simulink model "pfb_fft_d3a"  (R2021a)
settings: Solver=VariableStepAuto  StartTime=0.0  StopTime=100.0  RelTol=1e-3
undefined symbols (not defined in the file): i, pfb_coeff_gen_calc
libraries: xbsIndex_r4 x11529, casper_library_misc x39, casper_library_delays x39, xbsReplacements_r4 x2
(part 1 of 118)
settings Model: Creator=tbuser  LastModifiedBy=ih

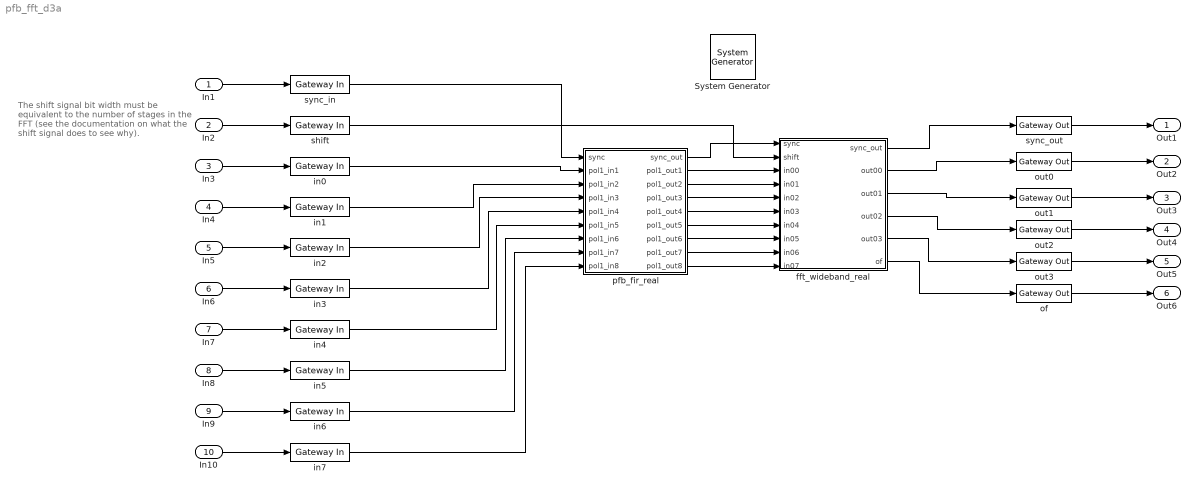
== system pfb_fft_d3a ==
  note: The shift signal bit width must be equivalent to the number of stages in the FFT (see the documentation on what the shift signal does to see why).
  In1 : Inport
  In2 : Inport  Port=2
  In3 : Inport  Port=3
  In4 : Inport  Port=4
  In5 : Inport  Port=5
  In6 : Inport  Port=6
  In7 : Inport  Port=7
  In8 : Inport  Port=8
  In9 : Inport  Port=9
  In10 : Inport  Port=10
  " System Generator" : xbsIndex_r4/ System Generator  Tag=genX  xilinxfamily=zynquplusRFSOC  part=xczu48dr  speed=-1-i  package=ffvg1517  synthesis_tool=Vivado  clock_wrapper=Clock Enables  directory=/home/ih/casper/pfb_fft_d3a  proj_type=Vivado  Synth_file=Vivado Synthesis Defaults  Impl_file=Vivado Implementation Defaults  testbench=off  simulink_period=1  sysclk_period=2.5  dcm_input_clock_period=10  incr_netlist=off  trim_vbits=Everywhere in SubSystem  dbl_ovrd=According to Block Masks  core_generation=According to Block Masks  run_coregen=off  deprecated_control=off  eval_field=0  block_type=sysgen
  fft_wideband_real : Subsystem  Tag=casper:fft_wideband_real  AncestorBlock=casper_library_ffts/fft_wideband_real  mask(fft_wideband_real){n_streams=1, FFTSize=14, n_inputs=3, input_bit_width=18, bin_pt_in=17, coeff_bit_width=18, unscramble=on, async=off, floating_point=off, float_type=single, exp_width=8, frac_width=24, add_latency=1, mult_latency=2, bram_latency=2, conv_latency=1, input_latency=0, biplex_direct_latency=0, add_pipe_latency=0, mult_pipe_latency=0, quantization=Round  (unbiased: Even Values), overflow=Wrap, delays_bit_limit=9, coeffs_bit_limit=9, coeff_sharing=on, coeff_decimation=on, coeff_generation=on, cal_bits=1, n_bits_rotation=25, mult_spec=2, max_fanout=4, bitgrowth=off, max_bits=18, hardcode_shifts=off, shift_schedule=[], dsp48_adders=off}
      mask prompts: n_streams "Number simultaneous streams"; FFTSize "Size of FFT: (2^? pts)"; n_inputs "Number of Simultaneous Inputs: (2^?)"; input_bit_width "Input Bit Width"; bin_pt_in "Input binary point"; coeff_bit_width "Coefficient Bit Width"; unscramble "Unscramble output (ie, put channels in canonical order)"; async "Asynchronous operation"; floating_point "floating point"; float_type "float type"; exp_width "exponent width"; frac_width "fraction width"; add_latency "Add Latency"; mult_latency "Mult Latency"; bram_latency "BRAM Latency"; conv_latency "Convert Latency"; input_latency "Input Latency"; biplex_direct_latency "Latency between biplexes and fft_direct"; add_pipe_latency "Add Interface Pipeline Latency"; mult_pipe_latency "CMult Pipeline Latency"; quantization "Quantization Behavior"; overflow "Overflow Behavior"; delays_bit_limit "Number bits above which to store stage's delays in BRAM (2^? bits)"; coeffs_bit_limit "Number bits above which to store stage's coefficients in BRAM (2^? bits)"; coeff_sharing "BRAM sharing in coeff storage"; coeff_decimation "Store a fraction of coeff factors where useful"; coeff_generation "Generate coeffs with multipliers where useful"; cal_bits "Number calibration locations when generating coeffs (2^?)"; n_bits_rotation "Feedback rotation vector resolution"; mult_spec "Multiplier impl. (0=core, 1=embedded, 2=behavioural) (left=1st stage, or just one value)"; max_fanout "Maximum fanout"; bitgrowth "Bitgrowth instead of shifting"; max_bits "Max bits to grow to"; hardcode_shifts "Hardcode shift schedule"; shift_schedule "Shift schedule"; dsp48_adders "DSP48 adders in butterfly"
      mask help: A real-sampled wideband FFT.
      mask init:
      | fft_wideband_real_init(gcb, ...
      |     'n_streams', n_streams, ...
      |     'FFTSize', FFTSize, ...
      |     'n_inputs', n_inputs, ...
      |     'input_bit_width', input_bit_width, ...
      |     'bin_pt_in', bin_pt_in, ...
      |     'coeff_bit_width', coeff_bit_width, ...
      |     'floating_point', floating_point, ...
      |     'float_type', float_type, ...
      |     'exp_width', exp_width, ...
      |     'frac_width', frac_width, ...
      |     'unscramble', unscramble, ...
      |     'async', async, ...
      |     'add_latency', add_latency, ...
      |     'mult_latency', mult_latency, ...
      |     'bram_latency', bram_latency, ...
      |     'conv_latency', conv_latency, ...
      |     'input_latency', input_latency, ...
      |     'add_pipe_latency', add_pipe_latency, ...
      |     'mult_pipe_latency', mult_pipe_latency, ...
      |     'biplex_direct_latency', biplex_direct_latency, ...
      |     'quantization', quantization, ...
      |     'overflow', overflow, ...
      |     'delays_bit_limit', delays_bit_limit, ...
      |     'coeffs_bit_limit', coeffs_bit_limit, ...
      |     'coeff_sharing', coeff_sharing, ...
      |     'coeff_decimation', coeff_decimation, ...
      |     'coeff_generation', coeff_generation, ...
      |     'cal_bits', cal_bits, ...
      |     'n_bits_rotation', n_bits_rotation, ...
      |     'max_fanout', max_fanout, ...   
      |     'mult_spec', mult_spec, ...
      |     'bitgrowth', bitgrowth, ...
      |     'max_bits', max_bits, ...
      |     'hardcode_shifts', hardcode_shifts, ...
      |     'shift_schedule', shift_schedule, ...
      |     'dsp48_adders', dsp48_adders);
      settings: AttributesFormatString=|
      | 14 stages
      | (18,18)
      | Round  (unbiased: Even Values)
      | Wrap
      mask Help: eval('xlWeb(''http://casper.berkeley.edu/wiki/Fft_wideband_real'')')
      mask Callback floating_point:
      | onoff = get_param(gcb, 'floating_point');
      | if strcmp(onoff,'on')
      |     enable_fixpt = 'off';
      |     set_param_state(gcb, 'float_type', 'on')
      | 
      |     f_type = get_param(gcb, 'float_type')
      |     if strcmp(f_type,'custom')
      |         set_param_state(gcb, 'exp_width', 'on')
      |         set_param_state(gcb, 'frac_width', 'on')
      |     else
      |         set_param_state(gcb, 'exp_width', 'off')
      |         set_param_state(gcb, 'frac_width', 'off')
      |     end
      | 
      | 
      | else
      |     enable_fixpt = 'on';
      |     set_param_state(gcb, 'float_type', 'off')
      |     set_param_state(gcb, 'exp_width', 'off')
      |     set_param_state(gcb, 'frac_width', 'off')
      | end
      | 
      | set_param_state(gcb, 'input_bit_width', enable_fixpt)
      | set_param_state(gcb, 'bin_pt_in', enable_fixpt)
      | set_param_state(gcb, 'coeff_bit_width', enable_fixpt)
      mask TypeOptions float_type: single | custom
      mask Callback float_type:
      | f_type = get_param(gcb, 'float_type');
      | if strcmp(f_type,'custom')
      |     set_param_state(gcb, 'exp_width', 'on')
      |     set_param_state(gcb, 'frac_width', 'on')
      | else
      |     set_param_state(gcb, 'exp_width', 'off')
      |     set_param_state(gcb, 'frac_width', 'off')
      | end
      mask TypeOptions quantization: Truncate | Round  (unbiased: +/- Inf) | Round  (unbiased: Even Values)
      mask TypeOptions overflow: Wrap | Saturate | Error
      mask Callback hardcode_shifts:
      | hardcode_shifts = get_param(gcb, 'hardcode_shifts');
      | set_param_state(gcb, 'shift_schedule', hardcode_shifts);
      mask Callback dsp48_adders: fft_callback_dsp48_adders(gcb);
      mask DialogControl ParameterTabVar0 Prompt: Basic
      mask DialogControl ParameterTabVar01 Prompt: Latency
      mask DialogControl ParameterTabVar012 Prompt: Implementation
  in{0..7} (8 alike) : xbsIndex_r4/Gateway In  gui_display_data_type=Fixed-point  arith_type="Signed  (2's comp)"  n_bits=14  bin_pt=0  preci_type=Single  exp_width=8  frac_width=24  rows=1  columns=1  quantization="Round  (unbiased: +/- Inf)"  overflow=Saturate  period=1  UseAsADC=off  ADCChannel='1'  interface=None  automatic_assignment=on  address_offset=hex2dec('00')  intf_name=''  intf_description=''  default_value=0  timing_constraint=None  locs_specified=off  LOCs={}  io_standard={}  inherit_from_input=off  hdl_port=on  dbl_ovrd=off  block_type=gatewayin
  of : xbsIndex_r4/Gateway Out  inherit_from_input=off  hdl_port=on  rows=1  columns=1  UseAsDAC=off  DACChannel='1'  interface=None  automatic_assignment=on  address_offset=hex2dec('00')  intf_name=''  intf_description=''  timing_constraint=None  locs_specified=off  LOCs={}  io_standard={}  block_type=gatewayout
  out{0..3} (4 alike) : xbsIndex_r4/Gateway Out  inherit_from_input=on  hdl_port=on  rows=1  columns=1  UseAsDAC=off  DACChannel='1'  interface=None  automatic_assignment=on  address_offset=hex2dec('00')  intf_name=''  intf_description=''  timing_constraint=None  locs_specified=off  LOCs={}  io_standard={}  block_type=gatewayout
  pfb_fir_real : Subsystem  Tag=casper:pfb_fir_real  AncestorBlock=casper_library_pfbs/pfb_fir_real  mask(pfb_fir_real){PFBSize=14, TotalTaps=4, WindowType=hamming, n_inputs=3, n_pol_blocks=1, MakeBiplex=off, BitWidthIn=14, BitWidthOut=18, CoeffBitWidth=18, CoeffDistMem=off, add_latency=1, mult_latency=2, bram_latency=2, fan_latency=1, conv_latency=1, quantization=Round  (unbiased: Even Values), fwidth=1, mult_spec=2, adder_folding=on, adder_imp=Fabric, coeffs_share=off}
      mask prompts: PFBSize "Size of PFB: (2^? pnts)"; TotalTaps "Total Number of Taps:"; WindowType "Windowing Function:"; n_inputs "Number of Simultaneous Inputs: (2^?)"; n_pol_blocks "Number of independent input streams (I.e., number of different polarizations)"; MakeBiplex "Make Biplex?"; BitWidthIn "Input Bitwidth:"; BitWidthOut "Output Bitwidth:"; CoeffBitWidth "Coefficient Bitwidth:"; CoeffDistMem "Use Distributed Memory for Coeffs"; add_latency "Add Latency"; mult_latency "Mult Latency"; bram_latency "BRAM Latency"; fan_latency "Fanout latency"; conv_latency "Convert latency"; quantization "Quantization Behavior"; fwidth "Bin Width Scaling (normal=1)"; mult_spec "Multiplier specification (0=core, 1=embedded, 2=behavioural) (left=1st tap, or just one value)"; adder_folding "Fold adders into DSPs"; adder_imp "Adder implementation"; coeffs_share "Share coefficients between polarisations (use less BRAM)?"
      mask help:
      | Fold adders into DSPs: Causes adders to be absorbed into DSP blocks (supported in Virtex5)
      | Adder implementation: Cores using Fabric or DSP48 or behavioral HDL
      mask init:
      | pfb_fir_real_init(gcb, ...
      |     'PFBSize', PFBSize, ...
      |     'TotalTaps', TotalTaps, ...
      |     'WindowType', WindowType, ...
      |     'n_inputs', n_inputs, ...
      |     'MakeBiplex', MakeBiplex, ...
      |     'BitWidthIn', BitWidthIn, ...
      |     'BitWidthOut', BitWidthOut, ...
      |     'CoeffBitWidth', CoeffBitWidth, ...
      |     'CoeffDistMem', CoeffDistMem, ...
      |     'add_latency', add_latency, ...
      |     'mult_latency', mult_latency, ...
      |     'bram_latency', bram_latency, ...
      |     'fan_latency', fan_latency, ...
      |     'conv_latency', conv_latency, ...
      |     'quantization', quantization, ...
      |     'fwidth', fwidth, ...
      |     'mult_spec', mult_spec, ...
      |     'adder_folding', adder_folding, ...
      |     'adder_imp', adder_imp, ...
      |     'coeffs_share', coeffs_share);
      settings: AttributesFormatString=taps=4, add_latency=1
      mask Help: eval('xlWeb(''http://casper.berkeley.edu/wiki/Pfb_fir_real'')')
      mask Callback TotalTaps:
      | %num_taps = eval(get_param(gcb, 'TotalTaps'));
      | %old_vec = eval(get_param(gcb, 'mult_spec'));=-0l
      | 
      | %vec = 2.*ones(1,num_taps);
      | %old_size = length(old_vec);
      | 
      | %if(old_size <= num_taps),
      | %    new_size = old_size;
      | %else,
      | %    new_size = num_taps;
      | %end
      | 
      | %for n = 1:new_size, vec(n) = old_vec(n); end
      | %set_param(gcb, 'mult_spec', mat2str(vec));
      mask TypeOptions WindowType: bartlett | barthannwin | blackman | blackmanharris | bohamwin | chebwin | flattopwin | gausswin | hamming | hann | kaiser | nuttallwin | parzenwin | rectwin | tukeywin | triang | userwindow
      mask TypeOptions quantization: Truncate | Round  (unbiased: +/- Inf) | Round  (unbiased: Even Values)
      mask TypeOptions adder_imp: Behavioral | Fabric | DSP48
  shift : xbsIndex_r4/Gateway In  gui_display_data_type=Fixed-point  arith_type=Unsigned  n_bits=14  bin_pt=0  preci_type=Single  exp_width=8  frac_width=24  rows=1  columns=1  quantization="Round  (unbiased: +/- Inf)"  overflow=Saturate  period=1  UseAsADC=off  ADCChannel='1'  interface=None  automatic_assignment=on  address_offset=hex2dec('00')  intf_name=''  intf_description=''  default_value=0  timing_constraint=None  locs_specified=off  LOCs={}  io_standard={}  inherit_from_input=off  hdl_port=on  dbl_ovrd=off  block_type=gatewayin
  sync_in : xbsIndex_r4/Gateway In  gui_display_data_type=Boolean  arith_type=Boolean  n_bits=16  bin_pt=14  preci_type=Single  exp_width=8  frac_width=24  rows=1  columns=1  quantization="Round  (unbiased: +/- Inf)"  overflow=Saturate  period=1  UseAsADC=off  ADCChannel='1'  interface=None  automatic_assignment=on  address_offset=hex2dec('00')  intf_name=''  intf_description=''  default_value=0  timing_constraint=None  locs_specified=off  LOCs={}  io_standard={}  inherit_from_input=off  hdl_port=on  dbl_ovrd=off  block_type=gatewayin
  sync_out : xbsIndex_r4/Gateway Out  inherit_from_input=off  hdl_port=on  rows=1  columns=1  UseAsDAC=off  DACChannel='1'  interface=None  automatic_assignment=on  address_offset=hex2dec('00')  intf_name=''  intf_description=''  timing_constraint=None  locs_specified=off  LOCs={}  io_standard={}  block_type=gatewayout
  Out1 : Outport
  Out2 : Outport  Port=2
  Out3 : Outport  Port=3
  Out4 : Outport  Port=4
  Out5 : Outport  Port=5
  Out6 : Outport  Port=6
  wires:
  fft_wideband_real/1(sync_out) -> sync_out/1
  fft_wideband_real/2(out00) -> out0/1
  fft_wideband_real/3(out01) -> out1/1
  fft_wideband_real/6(of) -> of/1
  fft_wideband_real/4(out02) -> out2/1
  fft_wideband_real/5(out03) -> out3/1
  pfb_fir_real/2(pol1_out1) -> fft_wideband_real/3(in00)
  pfb_fir_real/3(pol1_out2) -> fft_wideband_real/4(in01)
  pfb_fir_real/4(pol1_out3) -> fft_wideband_real/5(in02)
  pfb_fir_real/5(pol1_out4) -> fft_wideband_real/6(in03)
  pfb_fir_real/6(pol1_out5) -> fft_wideband_real/7(in04)
  pfb_fir_real/7(pol1_out6) -> fft_wideband_real/8(in05)
  pfb_fir_real/8(pol1_out7) -> fft_wideband_real/9(in06)
  pfb_fir_real/9(pol1_out8) -> fft_wideband_real/10(in07)
  shift/1 -> fft_wideband_real/2(shift)
  sync_in/1 -> pfb_fir_real/1(sync)
  pfb_fir_real/1(sync_out) -> fft_wideband_real/1(sync)
  in0/1 -> pfb_fir_real/2(pol1_in1)
  in1/1 -> pfb_fir_real/3(pol1_in2)
  in2/1 -> pfb_fir_real/4(pol1_in3)
  in3/1 -> pfb_fir_real/5(pol1_in4)
  in4/1 -> pfb_fir_real/6(pol1_in5)
  in5/1 -> pfb_fir_real/7(pol1_in6)
  in6/1 -> pfb_fir_real/8(pol1_in7)
  in7/1 -> pfb_fir_real/9(pol1_in8)
  In1/1 -> sync_in/1
  In2/1 -> shift/1
  In3/1 -> in0/1
  In4/1 -> in1/1
  In5/1 -> in2/1
  In6/1 -> in3/1
  In7/1 -> in4/1
  In8/1 -> in5/1
  In9/1 -> in6/1
  In10/1 -> in7/1
  sync_out/1 -> Out1/1
  out0/1 -> Out2/1
  out1/1 -> Out3/1
  out2/1 -> Out4/1
  out3/1 -> Out5/1
  of/1 -> Out6/1

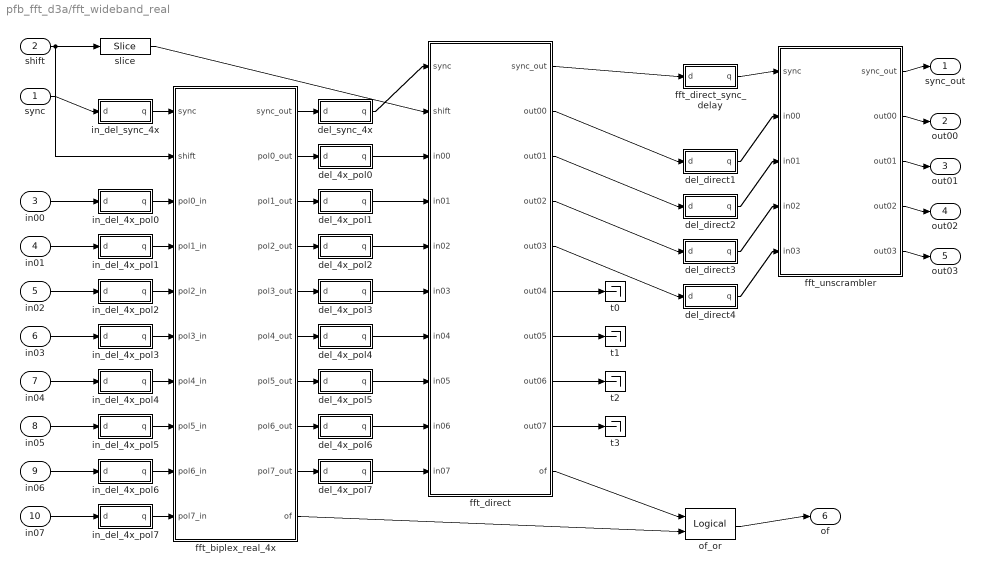
== system pfb_fft_d3a/fft_wideband_real ==
  sync : Inport
  shift : Inport  Port=2
  in00 : Inport  Port=3
  in01 : Inport  Port=4
  in02 : Inport  Port=5
  in03 : Inport  Port=6
  in04 : Inport  Port=7
  in05 : Inport  Port=8
  in06 : Inport  Port=9
  in07 : Inport  Port=10
  del_4x_pol0 : Subsystem  AncestorBlock=casper_library_delays/pipeline  mask(pipeline){csp_latency=0}
      mask prompts: csp_latency "Latency"
      mask help:
      | An explicitly laid-out delay line to avoid mapping to SRL16s
      | for use in pipelining to help achieve timing closure.
      mask init:
      | pipeline_init(gcb,'latency',csp_latency);
      settings: AttributesFormatString=Latency = %<latency>
      mask Display:
      | port_label('input', 1, 'd');
      | port_label('output', 1, 'q');
      | disp(['Z^-', num2str(csp_latency)]);
  del_4x_pol1 : Subsystem  AncestorBlock=casper_library_delays/pipeline  mask(pipeline){csp_latency=0}
      mask prompts: csp_latency "Latency"
      mask help:
      | An explicitly laid-out delay line to avoid mapping to SRL16s
      | for use in pipelining to help achieve timing closure.
      mask init:
      | pipeline_init(gcb,'latency',csp_latency);
      settings: AttributesFormatString=Latency = %<latency>
      mask Display:
      | port_label('input', 1, 'd');
      | port_label('output', 1, 'q');
      | disp(['Z^-', num2str(csp_latency)]);
  del_4x_pol2 : Subsystem  AncestorBlock=casper_library_delays/pipeline  mask(pipeline){csp_latency=0}
      mask prompts: csp_latency "Latency"
      mask help:
      | An explicitly laid-out delay line to avoid mapping to SRL16s
      | for use in pipelining to help achieve timing closure.
      mask init:
      | pipeline_init(gcb,'latency',csp_latency);
      settings: AttributesFormatString=Latency = %<latency>
      mask Display:
      | port_label('input', 1, 'd');
      | port_label('output', 1, 'q');
      | disp(['Z^-', num2str(csp_latency)]);
  del_4x_pol3 : Subsystem  AncestorBlock=casper_library_delays/pipeline  mask(pipeline){csp_latency=0}
      mask prompts: csp_latency "Latency"
      mask help:
      | An explicitly laid-out delay line to avoid mapping to SRL16s
      | for use in pipelining to help achieve timing closure.
      mask init:
      | pipeline_init(gcb,'latency',csp_latency);
      settings: AttributesFormatString=Latency = %<latency>
      mask Display:
      | port_label('input', 1, 'd');
      | port_label('output', 1, 'q');
      | disp(['Z^-', num2str(csp_latency)]);
  del_4x_pol4 : Subsystem  AncestorBlock=casper_library_delays/pipeline  mask(pipeline){csp_latency=0}
      mask prompts: csp_latency "Latency"
      mask help:
      | An explicitly laid-out delay line to avoid mapping to SRL16s
      | for use in pipelining to help achieve timing closure.
      mask init:
      | pipeline_init(gcb,'latency',csp_latency);
      settings: AttributesFormatString=Latency = %<latency>
      mask Display:
      | port_label('input', 1, 'd');
      | port_label('output', 1, 'q');
      | disp(['Z^-', num2str(csp_latency)]);
  del_4x_pol5 : Subsystem  AncestorBlock=casper_library_delays/pipeline  mask(pipeline){csp_latency=0}
      mask prompts: csp_latency "Latency"
      mask help:
      | An explicitly laid-out delay line to avoid mapping to SRL16s
      | for use in pipelining to help achieve timing closure.
      mask init:
      | pipeline_init(gcb,'latency',csp_latency);
      settings: AttributesFormatString=Latency = %<latency>
      mask Display:
      | port_label('input', 1, 'd');
      | port_label('output', 1, 'q');
      | disp(['Z^-', num2str(csp_latency)]);
  del_4x_pol6 : Subsystem  AncestorBlock=casper_library_delays/pipeline  mask(pipeline){csp_latency=0}
      mask prompts: csp_latency "Latency"
      mask help:
      | An explicitly laid-out delay line to avoid mapping to SRL16s
      | for use in pipelining to help achieve timing closure.
      mask init:
      | pipeline_init(gcb,'latency',csp_latency);
      settings: AttributesFormatString=Latency = %<latency>
      mask Display:
      | port_label('input', 1, 'd');
      | port_label('output', 1, 'q');
      | disp(['Z^-', num2str(csp_latency)]);
  del_4x_pol7 : Subsystem  AncestorBlock=casper_library_delays/pipeline  mask(pipeline){csp_latency=0}
      mask prompts: csp_latency "Latency"
      mask help:
      | An explicitly laid-out delay line to avoid mapping to SRL16s
      | for use in pipelining to help achieve timing closure.
      mask init:
      | pipeline_init(gcb,'latency',csp_latency);
      settings: AttributesFormatString=Latency = %<latency>
      mask Display:
      | port_label('input', 1, 'd');
      | port_label('output', 1, 'q');
      | disp(['Z^-', num2str(csp_latency)]);
  del_direct1 : Subsystem  AncestorBlock=casper_library_delays/pipeline  mask(pipeline){csp_latency=0}
      mask prompts: csp_latency "Latency"
      mask help:
      | An explicitly laid-out delay line to avoid mapping to SRL16s
      | for use in pipelining to help achieve timing closure.
      mask init:
      | pipeline_init(gcb,'latency',csp_latency);
      settings: AttributesFormatString=Latency = %<latency>
      mask Display:
      | port_label('input', 1, 'd');
      | port_label('output', 1, 'q');
      | disp(['Z^-', num2str(csp_latency)]);
  del_direct2 : Subsystem  AncestorBlock=casper_library_delays/pipeline  mask(pipeline){csp_latency=0}
      mask prompts: csp_latency "Latency"
      mask help:
      | An explicitly laid-out delay line to avoid mapping to SRL16s
      | for use in pipelining to help achieve timing closure.
      mask init:
      | pipeline_init(gcb,'latency',csp_latency);
      settings: AttributesFormatString=Latency = %<latency>
      mask Display:
      | port_label('input', 1, 'd');
      | port_label('output', 1, 'q');
      | disp(['Z^-', num2str(csp_latency)]);
  del_direct3 : Subsystem  AncestorBlock=casper_library_delays/pipeline  mask(pipeline){csp_latency=0}
      mask prompts: csp_latency "Latency"
      mask help:
      | An explicitly laid-out delay line to avoid mapping to SRL16s
      | for use in pipelining to help achieve timing closure.
      mask init:
      | pipeline_init(gcb,'latency',csp_latency);
      settings: AttributesFormatString=Latency = %<latency>
      mask Display:
      | port_label('input', 1, 'd');
      | port_label('output', 1, 'q');
      | disp(['Z^-', num2str(csp_latency)]);
  del_direct4 : Subsystem  AncestorBlock=casper_library_delays/pipeline  mask(pipeline){csp_latency=0}
      mask prompts: csp_latency "Latency"
      mask help:
      | An explicitly laid-out delay line to avoid mapping to SRL16s
      | for use in pipelining to help achieve timing closure.
      mask init:
      | pipeline_init(gcb,'latency',csp_latency);
      settings: AttributesFormatString=Latency = %<latency>
      mask Display:
      | port_label('input', 1, 'd');
      | port_label('output', 1, 'q');
      | disp(['Z^-', num2str(csp_latency)]);
  del_sync_4x : Subsystem  AncestorBlock=casper_library_delays/pipeline  mask(pipeline){csp_latency=0}
      mask prompts: csp_latency "Latency"
      mask help:
      | An explicitly laid-out delay line to avoid mapping to SRL16s
      | for use in pipelining to help achieve timing closure.
      mask init:
      | pipeline_init(gcb,'latency',csp_latency);
      settings: AttributesFormatString=Latency = %<latency>
      mask Display:
      | port_label('input', 1, 'd');
      | port_label('output', 1, 'q');
      | disp(['Z^-', num2str(csp_latency)]);
  fft_biplex_real_4x : Subsystem  Tag=casper:fft_biplex_real_4x  AncestorBlock=casper_library_ffts/fft_biplex_real_4x  mask(fft_biplex_real_4x){n_inputs=2, FFTSize=11, input_bit_width=18, bin_pt_in=17, coeff_bit_width=18, async=off, floating_point=off, float_type=single, exp_width=8, frac_width=24, add_latency=1, mult_latency=2, bram_latency=2, conv_latency=1, add_pipe_latency=0, mult_pipe_latency=0, quantization=Round  (unbiased: Even Values), overflow=Wrap, delays_bit_limit=9, coeffs_bit_limit=9, coeff_sharing=on, coeff_decimation=on, max_fanout=4, mult_spec=[2 2 2 2 2 2 2 2 2 2 2], bitgrowth=off, max_bits=18, hardcode_shifts=off, shift_schedule=[1 1 1 1 1 1 1 1 1 1 1], dsp48_adders=off}
      mask prompts: n_inputs "Number simultaneous inputs (4*?)"; FFTSize "Size of FFT: (2^? pts)"; input_bit_width "Input bit width"; bin_pt_in "Input binary point"; coeff_bit_width "Coefficient Bit Width"; async "Asynchronous operation"; floating_point "floating point"; float_type "float type"; exp_width "exponent width"; frac_width "fraction width"; add_latency "Add Latency"; mult_latency "Mult Latency"; bram_latency "BRAM Latency"; conv_latency "Convert latency"; add_pipe_latency "Add Interface Pipeline Latency"; mult_pipe_latency "CMult Pipeline Latency"; quantization "Quantization Behavior"; overflow "Overflow Behavior"; delays_bit_limit "Number bits above which to implement stage's delays in BRAM (2^? bits)"; coeffs_bit_limit "Number bits above which to store stage's coefficients in BRAM (2^? bits)"; coeff_sharing "BRAM sharing in coeff storage"; coeff_decimation "Store a fraction of coeff factors where useful"; max_fanout "Maximum fanout"; mult_spec "Multiplier impl. (0=core, 1=embedded, 2=behavioural) (left=1st stage, or just one value)"; bitgrowth "Bitgrowth instead of shifting"; max_bits "Max bits to grow to"; hardcode_shifts "Hardcode shift schedule"; shift_schedule "Shift schedule"; dsp48_adders "DSP48 adders in butterfly"
      mask help: A real-sampled biplex FFT, with output demuxed by 4.
      mask init:
      | fft_biplex_real_4x_init(gcb, ...
      |     'n_inputs', n_inputs, ...
      |     'FFTSize', FFTSize, ...
      |     'input_bit_width', input_bit_width, ...
      |     'bin_pt_in', bin_pt_in, ...
      |     'coeff_bit_width', coeff_bit_width, ...
      |     'floating_point', floating_point, ...
      |     'float_type', float_type, ...
      |     'exp_width', exp_width, ...
      |     'frac_width', frac_width, ...    
      |     'async', async, ...
      |     'add_latency', add_latency, ...
      |     'mult_latency', mult_latency, ...
      |     'bram_latency', bram_latency, ...
      |     'conv_latency', conv_latency, ...
      |     'add_pipe_latency', add_pipe_latency, ...
      |     'mult_pipe_latency', mult_pipe_latency, ...    
      |     'quantization', quantization, ...
      |     'overflow', overflow, ...
      |     'delays_bit_limit', delays_bit_limit, ... 
      |     'coeffs_bit_limit', coeffs_bit_limit, ...
      |     'coeff_sharing', coeff_sharing, ...
      |     'coeff_decimation', coeff_decimation, ...
      |     'max_fanout', max_fanout, ...   
      |     'mult_spec', mult_spec, ...
      |     'bitgrowth', bitgrowth, ...
      |     'max_bits', max_bits, ...
      |     'hardcode_shifts', hardcode_shifts, ...
      |     'shift_schedule', shift_schedule, ...
      |     'dsp48_adders', dsp48_adders);
      settings: AttributesFormatString=|
      | 11 stages
      | [18,18]
      | Round  (unbiased: Even Values)
      | Wrap
      mask Help: eval('xlWeb(''http://casper.berkeley.edu/wiki/Fft_biplex_real_4x'')')
      mask Callback floating_point:
      | onoff = get_param(gcb, 'floating_point');
      | if strcmp(onoff,'on')
      |     enable_fixpt = 'off'
      |     set_param_state(gcb, 'float_type', 'on')
      | 
      |     f_type = get_param(gcb, 'float_type')
      |     if strcmp(f_type,'custom')
      |        set_param_state(gcb, 'exp_width', 'on')
      |        set_param_state(gcb, 'frac_width', 'on')
      |     else
      |        set_param_state(gcb, 'exp_width', 'off')
      |        set_param_state(gcb, 'frac_width', 'off')
      |     end
      | 
      | 
      | else
      |     enable_fixpt = 'on'
      |     set_param_state(gcb, 'float_type', 'off')
      |     set_param_state(gcb, 'exp_width', 'off')
      |     set_param_state(gcb, 'frac_width', 'off')
      | end
      | 
      | set_param_state(gcb, 'input_bit_width', enable_fixpt)
      | set_param_state(gcb, 'bin_pt_in', enable_fixpt)
      | set_param_state(gcb, 'coeff_bit_width', enable_fixpt)
      mask TypeOptions float_type: single | custom
      mask Callback float_type:
      | f_type = get_param(gcb, 'float_type')
      | if strcmp(f_type,'custom')
      |     set_param_state(gcb, 'exp_width', 'on')
      |     set_param_state(gcb, 'frac_width', 'on')
      | else
      |     set_param_state(gcb, 'exp_width', 'off')
      |     set_param_state(gcb, 'frac_width', 'off')
      | end
      mask TypeOptions quantization: Truncate | Round  (unbiased: +/- Inf) | Round  (unbiased: Even Values)
      mask TypeOptions overflow: Wrap | Saturate | Error
      mask Callback hardcode_shifts:
      | hardcode_shifts = get_param(gcb, 'hardcode_shifts');
      | set_param_state(gcb, 'shift_schedule', hardcode_shifts);
      mask Callback dsp48_adders: fft_callback_dsp48_adders(gcb);
      mask DialogControl ParameterTabVar0 Prompt: Basic
      mask DialogControl ParameterTabVar01 Prompt: Latency
      mask DialogControl ParameterTabVar012 Prompt: Implementation
  fft_direct : Subsystem  AncestorBlock=casper_library_ffts/fft_direct  mask(fft_direct){n_streams=1, FFTSize=3, input_bit_width=18, bin_pt_in=17, coeff_bit_width=18, map_tail=on, LargerFFTSize=14, StartStage=12, async=off, floating_point=off, float_type=single, exp_width=8, frac_width=24, add_latency=1, mult_latency=2, bram_latency=2, conv_latency=1, add_pipe_latency=0, mult_pipe_latency=0, quantization=Round  (unbiased: Even Values), overflow=Wrap, coeffs_bit_limit=9, coeff_sharing=on, coeff_decimation=on, coeff_generation=on, cal_bits=1, n_bits_rotation=25, max_fanout=4, mult_spec=[2 2 2], bitgrowth=off, max_bits=18, hardcode_shifts=off, shift_schedule=[1 1 1], dsp48_adders=off}
      mask prompts: n_streams "Number simultaneous streams"; FFTSize "Size of FFT: (2^? pts)"; input_bit_width "Input Bit Width"; bin_pt_in "Input binary point"; coeff_bit_width "Coefficient Bit Width"; map_tail "Map Tail of Larger FFT"; LargerFFTSize "Size of Larger FFT (2^?)"; StartStage "Start Stage of Map Tail"; async "Asynchronous operation"; floating_point "floating point"; exp_width "exponent width"; frac_width "fraction width"; add_latency "Add Latency"; mult_latency "Mult Latency"; bram_latency "BRAM Latency"; conv_latency "Convert latency"; add_pipe_latency "Add interface pipeline latency"; mult_pipe_latency "Cmult pipeline latency"; quantization "Quantization Behavior"; overflow "Overflow Behavior"; coeffs_bit_limit "Number bits above which to store stage's coefficients in BRAM (2^? bits)"; coeff_sharing "BRAM sharing in coeff storage"; coeff_decimation "Store a fraction of coeff factors where useful"; coeff_generation "Generate coeffs with multipliers where useful"; cal_bits "Number calibration locations when generating coeffs (2^?)"; n_bits_rotation "Feedback rotation vector resolution"; max_fanout "Maximum fanout"; mult_spec "Multiplier impl. (0=core, 1=embedded, 2=behavioural) (left=1st stage, or just one value)"; bitgrowth "Bit growth instead of shifting"; max_bits "Max bits to growth to"; hardcode_shifts "Hardcode shift schedule"; shift_schedule "Shift schedule"; dsp48_adders "DSP48 adders in butterfly"
      mask help:
      | FFT internal block.
      |
      | Implements an N-point FFT as the classic butterfly structure,
      | with N inputs and N outputs.
      mask init:
      | fft_direct_init(gcb, ...
      |     'n_streams', n_streams, ...
      |     'FFTSize', FFTSize, ...
      |     'input_bit_width', input_bit_width, ...
      |     'bin_pt_in', bin_pt_in, ...
      |     'coeff_bit_width', coeff_bit_width, ...
      |     'map_tail', map_tail, ...
      |     'LargerFFTSize', LargerFFTSize, ...
      |     'StartStage', StartStage, ...
      |     'async', async, ...
      |     'add_latency', add_latency, ...
      |     'mult_latency', mult_latency, ...
      |     'bram_latency', bram_latency, ...
      |     'conv_latency', conv_latency, ...
      |     'add_pipe_latency', add_pipe_latency, ...
      |     'mult_pipe_latency', mult_pipe_latency, ...          
      |     'quantization', quantization, ...
      |     'overflow', overflow, ...
      |     'coeffs_bit_limit', coeffs_bit_limit, ...
      |     'coeff_sharing', coeff_sharing, ...
      |     'coeff_decimation', coeff_decimation, ...
      |     'coeff_generation', coeff_generation, ...
      |     'floating_point', floating_point, ...
      |     'float_type', float_type, ...
      |     'exp_width', exp_width, ...
      |     'frac_width', frac_width, ...      
      |     'cal_bits', cal_bits, ...
      |     'n_bits_rotation', n_bits_rotation, ...
      |     'max_fanout', max_fanout, ...
      |     'mult_spec', mult_spec, ...
      |     'bitgrowth', bitgrowth, ...
      |     'max_bits', max_bits, ...
      |     'hardcode_shifts', hardcode_shifts, ...
      |     'shift_schedule', shift_schedule, ...
      |     'dsp48_adders', dsp48_adders);
      settings: AttributesFormatString=|
      | stages [12:14] of 14
      | [18,18]
      | Round  (unbiased: Even Values)
      | Wrap
      mask Callback map_tail:
      | map_tail = get_param(gcb, 'map_tail');
      | set_param_state(gcb, 'LargerFFTSize', map_tail);
      | set_param_state(gcb, 'StartStage', map_tail);
      mask Callback floating_point:
      | onoff = get_param(gcb, 'floating_point');
      | if strcmp(onoff,'on')
      |     enable_fixpt = 'off';
      |     set_param_state(gcb, 'float_type', 'on')
      | 
      |     f_type = get_param(gcb, 'float_type');
      |     if strcmp(f_type,'custom')
      |         set_param_state(gcb, 'exp_width', 'on')
      |         set_param_state(gcb, 'frac_width', 'on')
      |     else
      |         set_param_state(gcb, 'exp_width', 'off')
      |         set_param_state(gcb, 'frac_width', 'off')
      |     end
      | 
      | 
      | else
      |     enable_fixpt = 'on';
      |     set_param_state(gcb, 'float_type', 'off')
      |     set_param_state(gcb, 'exp_width', 'off')
      |     set_param_state(gcb, 'frac_width', 'off')
      | end
      | 
      | set_param_state(gcb, 'input_bit_width', enable_fixpt)
      | set_param_state(gcb, 'bin_pt_in', enable_fixpt)
      | set_param_state(gcb, 'coeff_bit_width', enable_fixpt)
      mask TypeOptions float_type: single | custom
      mask Callback float_type:
      | f_type = get_param(gcb, 'float_type');
      | if strcmp(f_type,'custom')
      |     set_param_state(gcb, 'exp_width', 'on')
      |     set_param_state(gcb, 'frac_width', 'on')
      | else
      |     set_param_state(gcb, 'exp_width', 'off')
      |     set_param_state(gcb, 'frac_width', 'off')
      | end
      mask TypeOptions quantization: Truncate | Round  (unbiased: +/- Inf) | Round  (unbiased: Even Values)
      mask TypeOptions overflow: Wrap | Saturate | Error
      mask Callback hardcode_shifts:
      | hardcode_shifts = get_param(gcb, 'hardcode_shifts');
      | set_param_state(gcb, 'shift_schedule', hardcode_shifts);
      mask Callback dsp48_adders: fft_callback_dsp48_adders(gcb);
      mask DialogControl ParameterTabVar0 Prompt: Basic
      mask DialogControl ParameterTabVar01 Prompt: Latency
      mask DialogControl ParameterTabVar012 Prompt: Implementation
  fft_direct_sync_delay : Subsystem  AncestorBlock=casper_library_delays/pipeline  mask(pipeline){csp_latency=0}
      mask prompts: csp_latency "Latency"
      mask help:
      | An explicitly laid-out delay line to avoid mapping to SRL16s
      | for use in pipelining to help achieve timing closure.
      mask init:
      | pipeline_init(gcb,'latency',csp_latency);
      settings: AttributesFormatString=Latency = %<latency>
      mask Display:
      | port_label('input', 1, 'd');
      | port_label('output', 1, 'q');
      | disp(['Z^-', num2str(csp_latency)]);
  fft_unscrambler : Subsystem  AncestorBlock=casper_library_ffts/fft_unscrambler  mask(fft_unscrambler){n_streams=1, FFTSize=13, n_inputs=2, n_bits_in=18, bram_latency=2, coeffs_bit_limit=9, async=off, floating_point=off, float_type=single, exp_width=8, frac_width=24}
      mask prompts: n_streams "Number of simultaneous streams"; FFTSize "Size of FFT: (2^?)"; n_inputs "Number of simultaneous inputs: (2^?)"; n_bits_in "Input bit width"; bram_latency "BRAM Latency"; coeffs_bit_limit "Number bits above which to store map coefficients in BRAM (2^? bits)"; async "Asynchronous operation"; floating_point "floating point"; float_type "float type"; exp_width "exponent width"; frac_width "fraction width"
      mask init:
      | fft_unscrambler_init(gcb, ...
      |     'n_streams', n_streams, ...
      |     'FFTSize',FFTSize, ... 
      |     'n_inputs', n_inputs, ...
      |     'n_bits_in', n_bits_in, ...
      |     'floating_point', floating_point, ...
      |     'float_type', float_type, ...
      |     'exp_width', exp_width, ...
      |     'frac_width', frac_width, ...    
      |     'bram_latency', bram_latency, ...
      |     'coeffs_bit_limit', coeffs_bit_limit, ...
      |     'async', async);
      settings: AttributesFormatString=FFTSize=13, n_inputs=2
      mask Callback floating_point:
      | onoff = get_param(gcb, 'floating_point');
      | if strcmp(onoff,'on')
      |     enable_fixpt = 'off';
      |     set_param_state(gcb, 'float_type', 'on')
      | 
      |     f_type = get_param(gcb, 'float_type');
      |     if strcmp(f_type,'custom')
      |         set_param_state(gcb, 'exp_width', 'on')
      |         set_param_state(gcb, 'frac_width', 'on')
      |     else
      |         set_param_state(gcb, 'exp_width', 'off')
      |         set_param_state(gcb, 'frac_width', 'off')
      |     end
      | 
      | 
      | else
      |     enable_fixpt = 'on';
      |     set_param_state(gcb, 'float_type', 'off')
      |     set_param_state(gcb, 'exp_width', 'off')
      |     set_param_state(gcb, 'frac_width', 'off')
      | end
      | 
      | set_param_state(gcb, 'n_bits_in', enable_fixpt)
      mask TypeOptions float_type: single | custom
      mask Callback float_type:
      | f_type = get_param(gcb, 'float_type');
      | if strcmp(f_type,'custom')
      |     set_param_state(gcb, 'exp_width', 'on')
      |     set_param_state(gcb, 'frac_width', 'on')
      | else
      |     set_param_state(gcb, 'exp_width', 'off')
      |     set_param_state(gcb, 'frac_width', 'off')
      | end
  in_del_4x_pol0 : Subsystem  AncestorBlock=casper_library_delays/pipeline  mask(pipeline){csp_latency=0}
      mask prompts: csp_latency "Latency"
      mask help:
      | An explicitly laid-out delay line to avoid mapping to SRL16s
      | for use in pipelining to help achieve timing closure.
      mask init:
      | pipeline_init(gcb,'latency',csp_latency);
      settings: AttributesFormatString=Latency = %<latency>
      mask Display:
      | port_label('input', 1, 'd');
      | port_label('output', 1, 'q');
      | disp(['Z^-', num2str(csp_latency)]);
  in_del_4x_pol1 : Subsystem  AncestorBlock=casper_library_delays/pipeline  mask(pipeline){csp_latency=0}
      mask prompts: csp_latency "Latency"
      mask help:
      | An explicitly laid-out delay line to avoid mapping to SRL16s
      | for use in pipelining to help achieve timing closure.
      mask init:
      | pipeline_init(gcb,'latency',csp_latency);
      settings: AttributesFormatString=Latency = %<latency>
      mask Display:
      | port_label('input', 1, 'd');
      | port_label('output', 1, 'q');
      | disp(['Z^-', num2str(csp_latency)]);
  in_del_4x_pol2 : Subsystem  AncestorBlock=casper_library_delays/pipeline  mask(pipeline){csp_latency=0}
      mask prompts: csp_latency "Latency"
      mask help:
      | An explicitly laid-out delay line to avoid mapping to SRL16s
      | for use in pipelining to help achieve timing closure.
      mask init:
      | pipeline_init(gcb,'latency',csp_latency);
      settings: AttributesFormatString=Latency = %<latency>
      mask Display:
      | port_label('input', 1, 'd');
      | port_label('output', 1, 'q');
      | disp(['Z^-', num2str(csp_latency)]);
  in_del_4x_pol3 : Subsystem  AncestorBlock=casper_library_delays/pipeline  mask(pipeline){csp_latency=0}
      mask prompts: csp_latency "Latency"
      mask help:
      | An explicitly laid-out delay line to avoid mapping to SRL16s
      | for use in pipelining to help achieve timing closure.
      mask init:
      | pipeline_init(gcb,'latency',csp_latency);
      settings: AttributesFormatString=Latency = %<latency>
      mask Display:
      | port_label('input', 1, 'd');
      | port_label('output', 1, 'q');
      | disp(['Z^-', num2str(csp_latency)]);
  in_del_4x_pol4 : Subsystem  AncestorBlock=casper_library_delays/pipeline  mask(pipeline){csp_latency=0}
      mask prompts: csp_latency "Latency"
      mask help:
      | An explicitly laid-out delay line to avoid mapping to SRL16s
      | for use in pipelining to help achieve timing closure.
      mask init:
      | pipeline_init(gcb,'latency',csp_latency);
      settings: AttributesFormatString=Latency = %<latency>
      mask Display:
      | port_label('input', 1, 'd');
      | port_label('output', 1, 'q');
      | disp(['Z^-', num2str(csp_latency)]);
  in_del_4x_pol5 : Subsystem  AncestorBlock=casper_library_delays/pipeline  mask(pipeline){csp_latency=0}
      mask prompts: csp_latency "Latency"
      mask help:
      | An explicitly laid-out delay line to avoid mapping to SRL16s
      | for use in pipelining to help achieve timing closure.
      mask init:
      | pipeline_init(gcb,'latency',csp_latency);
      settings: AttributesFormatString=Latency = %<latency>
      mask Display:
      | port_label('input', 1, 'd');
      | port_label('output', 1, 'q');
      | disp(['Z^-', num2str(csp_latency)]);
  in_del_4x_pol6 : Subsystem  AncestorBlock=casper_library_delays/pipeline  mask(pipeline){csp_latency=0}
      mask prompts: csp_latency "Latency"
      mask help:
      | An explicitly laid-out delay line to avoid mapping to SRL16s
      | for use in pipelining to help achieve timing closure.
      mask init:
      | pipeline_init(gcb,'latency',csp_latency);
      settings: AttributesFormatString=Latency = %<latency>
      mask Display:
      | port_label('input', 1, 'd');
      | port_label('output', 1, 'q');
      | disp(['Z^-', num2str(csp_latency)]);
  in_del_4x_pol7 : Subsystem  AncestorBlock=casper_library_delays/pipeline  mask(pipeline){csp_latency=0}
      mask prompts: csp_latency "Latency"
      mask help:
      | An explicitly laid-out delay line to avoid mapping to SRL16s
      | for use in pipelining to help achieve timing closure.
      mask init:
      | pipeline_init(gcb,'latency',csp_latency);
      settings: AttributesFormatString=Latency = %<latency>
      mask Display:
      | port_label('input', 1, 'd');
      | port_label('output', 1, 'q');
      | disp(['Z^-', num2str(csp_latency)]);
  in_del_sync_4x : Subsystem  AncestorBlock=casper_library_delays/pipeline  mask(pipeline){csp_latency=0}
      mask prompts: csp_latency "Latency"
      mask help:
      | An explicitly laid-out delay line to avoid mapping to SRL16s
      | for use in pipelining to help achieve timing closure.
      mask init:
      | pipeline_init(gcb,'latency',csp_latency);
      settings: AttributesFormatString=Latency = %<latency>
      mask Display:
      | port_label('input', 1, 'd');
      | port_label('output', 1, 'q');
      | disp(['Z^-', num2str(csp_latency)]);
  of_or : xbsIndex_r4/Logical  logical_function=OR  inputs=2  en=off  latency=1  precision=Full  arith_type=Unsigned  n_bits=16  bin_pt=0  align_bp=on  dbl_ovrd=off  block_type=logical
  slice : xbsIndex_r4/Slice  nbits=3  boolean_output=off  mode=Lower Bit Location + Width  bit1=0  base1=MSB of Input  bit0=11  base0=LSB of Input  dbl_ovrd=off  block_type=slice
  t{0..3} (4 alike) : Terminator
  sync_out : Outport
  out00 : Outport  Port=2
  out01 : Outport  Port=3
  out02 : Outport  Port=4
  out03 : Outport  Port=5
  of : Outport  Port=6
  wires:
  sync/1 -> in_del_sync_4x/1(d)
  shift/1 -> fft_biplex_real_4x/2(shift), slice/1
  in_del_sync_4x/1(q) -> fft_biplex_real_4x/1(sync)
  fft_biplex_real_4x/1(sync_out) -> del_sync_4x/1(d)
  del_sync_4x/1(q) -> fft_direct/1(sync)
  fft_direct/6(out04) -> t0/1
  fft_direct/7(out05) -> t1/1
  fft_direct/8(out06) -> t2/1
  fft_direct/9(out07) -> t3/1
  fft_direct/1(sync_out) -> fft_direct_sync_delay/1(d)
  fft_direct_sync_delay/1(q) -> fft_unscrambler/1(sync)
  fft_unscrambler/1(sync_out) -> sync_out/1
  fft_direct/2(out00) -> del_direct1/1(d)
  del_direct1/1(q) -> fft_unscrambler/2(in00)
  fft_unscrambler/2(out00) -> out00/1
  fft_direct/3(out01) -> del_direct2/1(d)
  del_direct2/1(q) -> fft_unscrambler/3(in01)
  fft_unscrambler/3(out01) -> out01/1
  fft_direct/4(out02) -> del_direct3/1(d)
  del_direct3/1(q) -> fft_unscrambler/4(in02)
  fft_unscrambler/4(out02) -> out02/1
  fft_direct/5(out03) -> del_direct4/1(d)
  del_direct4/1(q) -> fft_unscrambler/5(in03)
  fft_unscrambler/5(out03) -> out03/1
  slice/1 -> fft_direct/2(shift)
  fft_biplex_real_4x/10(of) -> of_or/2
  fft_direct/10(of) -> of_or/1
  of_or/1 -> of/1
  in00/1 -> in_del_4x_pol0/1(d)
  in_del_4x_pol0/1(q) -> fft_biplex_real_4x/3(pol0_in)
  fft_biplex_real_4x/2(pol0_out) -> del_4x_pol0/1(d)
  del_4x_pol0/1(q) -> fft_direct/3(in00)
  in01/1 -> in_del_4x_pol1/1(d)
  in_del_4x_pol1/1(q) -> fft_biplex_real_4x/4(pol1_in)
  fft_biplex_real_4x/3(pol1_out) -> del_4x_pol1/1(d)
  del_4x_pol1/1(q) -> fft_direct/4(in01)
  in02/1 -> in_del_4x_pol2/1(d)
  in_del_4x_pol2/1(q) -> fft_biplex_real_4x/5(pol2_in)
  fft_biplex_real_4x/4(pol2_out) -> del_4x_pol2/1(d)
  del_4x_pol2/1(q) -> fft_direct/5(in02)
  in03/1 -> in_del_4x_pol3/1(d)
  in_del_4x_pol3/1(q) -> fft_biplex_real_4x/6(pol3_in)
  fft_biplex_real_4x/5(pol3_out) -> del_4x_pol3/1(d)
  del_4x_pol3/1(q) -> fft_direct/6(in03)
  in04/1 -> in_del_4x_pol4/1(d)
  in_del_4x_pol4/1(q) -> fft_biplex_real_4x/7(pol4_in)
  fft_biplex_real_4x/6(pol4_out) -> del_4x_pol4/1(d)
  del_4x_pol4/1(q) -> fft_direct/7(in04)
  in05/1 -> in_del_4x_pol5/1(d)
  in_del_4x_pol5/1(q) -> fft_biplex_real_4x/8(pol5_in)
  fft_biplex_real_4x/7(pol5_out) -> del_4x_pol5/1(d)
  del_4x_pol5/1(q) -> fft_direct/8(in05)
  in06/1 -> in_del_4x_pol6/1(d)
  in_del_4x_pol6/1(q) -> fft_biplex_real_4x/9(pol6_in)
  fft_biplex_real_4x/8(pol6_out) -> del_4x_pol6/1(d)
  del_4x_pol6/1(q) -> fft_direct/9(in06)
  in07/1 -> in_del_4x_pol7/1(d)
  in_del_4x_pol7/1(q) -> fft_biplex_real_4x/10(pol7_in)
  fft_biplex_real_4x/9(pol7_out) -> del_4x_pol7/1(d)
  del_4x_pol7/1(q) -> fft_direct/10(in07)
